simulink model "ref_multirate"  (R2026a)
settings: Solver=ode45  StopTime=1  FixedStep=1e-3  MaxStep=1e-2  RelTol=1e-10  AbsTol=1e-12
settings Model: Creator=djangovanderplas  LastModifiedBy=djangovanderplas
settings DataIOCC: OutputOption=SpecifiedOutputTimes  OutputTimes=0:1e-3:1

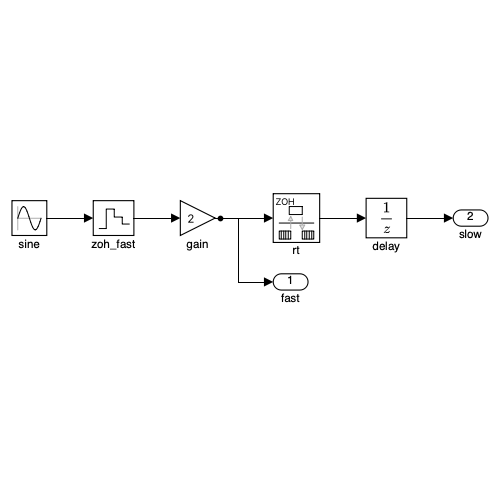
[thumbnail: Simulink's stored preview of the top-level diagram]
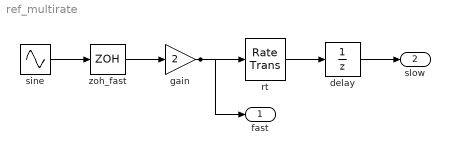
== system ref_multirate ==
  delay : UnitDelay  SampleTime=0.01
  gain : Gain  Gain=2
  rt : RateTransition  OutPortSampleTime=0.01
  sine : Sin  Frequency=2*pi  SampleTime=0
  zoh_fast : ZeroOrderHold  SampleTime=0.001
  fast : Outport
  slow : Outport  Port=2
  wires:
  rt/1 -> delay/1
  gain/1 -> fast/1, rt/1
  delay/1 -> slow/1
  zoh_fast/1 -> gain/1
  sine/1 -> zoh_fast/1
